simulink model "FMS"  (R2018b)
settings: configuration reference "fms_config" (kept outside this file)
values from neighbouring files (symbols this model uses):
  FMS_EXPORT = Simulink.Parameter(FMS_EXPORT_VALUE)    [fms_model_init.m]
  FMS_PARAM = Simulink.Parameter(FMS_PARAM_VALUE)    [fms_model_init.m]
undefined symbols (not defined in the file or in its folder): actuator_cmd, cmd_mask, ControlMode, ctrl_mode, DiscIntNeverNeededParam, FMS_Cmd, FMS_CONST, home, mode, PilotMode, r_cmd, reset, state, status, timestamp, u_cmd, VehicleState, VehicleStatus, wp_consume, wp_current
libraries: simulink x45, FMT_Model_Lib x35, hdlsllib x2
(part 2 of 3)

== system FMS/FMS Commander/Commander/Arm/Assist/Position/Position Command/Detect Movement ==
  FMS_In : Inport
  Abs1 : Abs
  Abs2 : Abs
  Bus Selector1 : BusSelector  OutputSignals=Pilot_Cmd.stick_roll,Pilot_Cmd.stick_throttle
  Compare To Constant : simulink/Logic and Bit Operations/Compare To Constant  relop=>  const=0.05  OutDataTypeStr=boolean
  Compare To Constant1 : simulink/Logic and Bit Operations/Compare To Constant  relop=<=  const=0.05  OutDataTypeStr=boolean
  Logical Operator : Logic  Operator=OR  AllPortsSameDT=off  OutDataTypeStr=boolean
  Motion State : Stateflow chart  TreatAsAtomicUnit=on
  motion_state : Outport
  wires:
  FMS_In/1 -> Bus Selector1/1
  Abs1/1 -> Compare To Constant/1
  Motion State/1(state) -> motion_state/1  "pos_ms"
  Bus Selector1/1 -> Abs1/1  "<stick_roll>"
  Compare To Constant1/1 -> Logical Operator/2
  Abs2/1 -> Compare To Constant1/1
  Bus Selector1/2 -> Abs2/1  "<stick_throttle>"
  Compare To Constant/1 -> Logical Operator/1
  Logical Operator/1 -> Motion State/1(motion_req)

== system FMS/FMS Commander/Commander/Arm/Assist/Position/Velocity_Command/DeadZone ==
  u : Inport
  Dead Zone : DeadZone  LowerValue=-th  UpperValue=th  SaturateOnIntegerOverflow=on
  Gain : Gain  Gain=1/(1-th)
  y : Outport
  wires:
  Gain/1 -> y/1
  Dead Zone/1 -> Gain/1
  u/1 -> Dead Zone/1

== system FMS/FMS Commander/Commander/Arm/Assist/Stabilize/Heading Command/Controller ==
  motion_state : Inport
  In Bus Element : Inport  Port=2  PortName=FMS_In
  In Bus Element1 : Inport  Port=2  PortName=FMS_In
  Brake Control : Subsystem  TreatAsAtomicUnit=on
  Hold Control : Subsystem  TreatAsAtomicUnit=on
  Merge : Merge  Inputs=3
  Move Control : Subsystem  TreatAsAtomicUnit=on
  Switch Case : SwitchCase  CaseConditions={MotionState.Hold, MotionState.Brake, MotionState.Move}  ShowDefaultCase=off
  psi_rate_cmd_radPs : Outport
  wires:
  Move Control/1(psi_rate_cmd_radPs) -> Merge/3
  Hold Control/1(psi_rate_cmd_radPs) -> Merge/1
  In Bus Element/1 -> Hold Control/1(FMS_In)
  Switch Case/1 -> Hold Control/Action
  motion_state/1 -> Switch Case/1
  In Bus Element1/1 -> Move Control/1(FMS_In)
  Merge/1 -> psi_rate_cmd_radPs/1
  Switch Case/3 -> Move Control/Action
  Brake Control/1(psi_rate_cmd_radPs) -> Merge/2
  Switch Case/2 -> Brake Control/Action

== system FMS/FMS Commander/Commander/Arm/Assist/Stabilize/Heading Command/Detect Movement ==
  FMS_In : Inport
  Abs1 : Abs
  Abs2 : Abs
  Bus Selector1 : BusSelector  OutputSignals=Pilot_Cmd.stick_roll,Pilot_Cmd.stick_throttle
  Compare To Constant : simulink/Logic and Bit Operations/Compare To Constant  relop=>  const=0.05  OutDataTypeStr=boolean
  Compare To Constant1 : simulink/Logic and Bit Operations/Compare To Constant  relop=<=  const=0.05  OutDataTypeStr=boolean
  Logical Operator : Logic  Operator=OR  AllPortsSameDT=off  OutDataTypeStr=boolean
  Motion State : Stateflow chart  TreatAsAtomicUnit=on
  motion_state : Outport
  wires:
  FMS_In/1 -> Bus Selector1/1
  Compare To Constant/1 -> Logical Operator/1
  Abs1/1 -> Compare To Constant/1
  Motion State/1(state) -> motion_state/1  "pos_ms"
  Bus Selector1/1 -> Abs1/1  "<stick_roll>"
  Bus Selector1/2 -> Abs2/1  "<stick_throttle>"
  Abs2/1 -> Compare To Constant1/1
  Compare To Constant1/1 -> Logical Operator/2
  Logical Operator/1 -> Motion State/1(motion_req)

== system FMS/FMS Commander/Commander/Arm/Auto/Mission/Mission_SubSystem/TD ==
  v : Inport
  Integrator : DiscreteIntegrator  SampleTime=-1  ICPrevOutput=DiscIntNeverNeededParam  ICPrevScaledInput=DiscIntNeverNeededParam
  Integrator1 : DiscreteIntegrator  SampleTime=-1  ICPrevOutput=DiscIntNeverNeededParam  ICPrevScaledInput=DiscIntNeverNeededParam
  Subtract : Sum  Inputs=+-
  "fhan " : Subsystem  mask{r0=2*9.806, h0=0.5}
      mask DialogControl ParameterGroupVar Prompt: fhan(v1,v2,r0,h0)
  v1 : Outport
  wires:
  "fhan "/1(fhan) -> Integrator/1
  Subtract/1 -> "fhan "/1(v1)
  Integrator/1 -> Integrator1/1, "fhan "/2(v2)  "v2"
  v/1 -> Subtract/2
  Integrator1/1 -> Subtract/1, v1/1

== system FMS/FMS Commander/Commander/Arm/Auto/Mission/Mission_SubSystem/Velocity Commander ==
  p1 : Inport
  p2 : Inport  Port=2
  p3 : Inport  Port=3
  L1 : Inport  Port=4
  In Bus Element : Inport  Port=5  PortName=FMS_In  Element=INS_Out.vn
  In Bus Element1 : Inport  Port=5  PortName=FMS_In  Element=INS_Out.ve
  AY_P : Gain  Gain=FMS_PARAM.AY_P
  L1 Reference WP : Subsystem
  Lateral Acceleration : Subsystem
  Mux1 : Mux  Inputs=2
  psi_rate_cmd : Outport
  wires:
  p3/1 -> Lateral Acceleration/3(p3), L1 Reference WP/3(P3)
  In Bus Element1/1 -> Mux1/2
  Mux1/1 -> Lateral Acceleration/1(Vg)
  p2/1 -> L1 Reference WP/2(P2)
  In Bus Element/1 -> Mux1/1
  L1 Reference WP/1(L1_WP) -> Lateral Acceleration/2(L1_WP)  "L1_WP"
  p1/1 -> L1 Reference WP/1(P1)
  L1/1 -> L1 Reference WP/4(L1), Lateral Acceleration/4(L1)
  Lateral Acceleration/1(l1_a_cmd) -> AY_P/1
  AY_P/1 -> psi_rate_cmd/1

== system FMS/FMS Commander/Commander/Arm/Auto/Mission/Mission_SubSystem/Way Points ==
  note: P1: path start point
      | P2: path end point
      | P3: vehicle point
  FMS_In : Inport
  Bus Selector : BusSelector  OutputSignals=INS_Out.x_R,INS_Out.y_R
  Bus Selector1 : BusSelector  OutputSignals=Cmd_In.sp_waypoint
  Bus Selector2 : BusSelector  OutputSignals=Cmd_In.cur_waypoint
  Mux : Mux  Inputs=2
  Reshape : Reshape  OutputDimensionality=Customize  OutputDimensions=[2,1]
  Reshape1 : Reshape  OutputDimensionality=Customize  OutputDimensions=[2,1]
  Reshape2 : Reshape  OutputDimensionality=Customize  OutputDimensions=[2,1]
  Selector : Selector  InputPortWidth=3  IndexOptions=Index vector (dialog)  Indices=[1 2]  OutputSizes=1
  Selector1 : Selector  InputPortWidth=3  IndexOptions=Index vector (dialog)  Indices=[1 2]  OutputSizes=1
  p1 : Outport
  p2 : Outport  Port=2
  p3 : Outport  Port=3
  wires:
  Reshape2/1 -> p3/1
  Reshape1/1 -> p1/1
  Reshape/1 -> p2/1
  Bus Selector/2 -> Mux/2  "<y_R>"
  Bus Selector/1 -> Mux/1  "<x_R>"
  Mux/1 -> Reshape2/1
  FMS_In/1 -> Bus Selector2/1, Bus Selector1/1, Bus Selector/1
  Bus Selector1/1 -> Selector/1  "<sp_waypoint>"
  Selector/1 -> Reshape/1
  Bus Selector2/1 -> Selector1/1  "<cur_waypoint>"
  Selector1/1 -> Reshape1/1

== system FMS/FMS Commander/Commander/Arm/Auto/Offboard/Rotation_Command/Heading_Control ==
  FMS_In : Inport
  Bus Selector1 : BusSelector  OutputSignals=Auto_Cmd.psi_cmd
  Bus Selector2 : BusSelector  OutputSignals=INS_Out.psi
  Gain2 : Gain  Gain=FMS_PARAM.YAW_P  OutDataTypeStr=single
  Sum : Sum  Inputs=-+|
  psi_err_saturation : Subsystem
  heading_r_cmd : Outport
  wires:
  Sum/1 -> psi_err_saturation/1(psi_err_in)  "psi_error_rad"
  psi_err_saturation/1(psi_err_rad) -> Gain2/1
  Gain2/1 -> heading_r_cmd/1
  FMS_In/1 -> Bus Selector1/1, Bus Selector2/1
  Bus Selector2/1 -> Sum/1  "<psi>"
  Bus Selector1/1 -> Sum/2  "<psi_cmd>"

== system FMS/FMS Commander/Commander/Arm/Auto/Offboard/Rotation_Command/Signal_Route ==
  FMS_In : Inport
  heading_r_cmd : Inport  Port=2
  pos_r_cmd : Inport  Port=3
  Bus Selector : BusSelector  OutputSignals=Auto_Cmd.cmd_mask
  Bus Selector1 : BusSelector  OutputSignals=Auto_Cmd.r_cmd
  Switch : Switch  Criteria=u2 > Threshold
  Switch1 : Switch  Criteria=u2 > Threshold
  psi_cmd_valid : simulink/Logic and Bit Operations/Bitwise Operator  logicop=AND  UseBitMask=on  BitMask=bin2dec('100000')  BitMaskRealWorld=Stored Integer
  r_cmd_valid : simulink/Logic and Bit Operations/Bitwise Operator  logicop=AND  UseBitMask=on  BitMask=bin2dec('100')  BitMaskRealWorld=Stored Integer
  r_cmd : Outport
  wires:
  FMS_In/1 -> Bus Selector1/1, Bus Selector/1
  pos_r_cmd/1 -> Switch1/3
  r_cmd_valid/1 -> Switch/2
  Bus Selector1/1 -> Switch/1  "<r_cmd>"
  Switch/1 -> r_cmd/1
  Bus Selector/1 -> psi_cmd_valid/1, r_cmd_valid/1  "<cmd_mask>"
  psi_cmd_valid/1 -> Switch1/2
  heading_r_cmd/1 -> Switch1/1
  Switch1/1 -> Switch/3

== system FMS/FMS Commander/Commander/Arm/Auto/Offboard/Rotation_Command/Velocity Commander ==
  p1 : Inport
  p2 : Inport  Port=2
  p3 : Inport  Port=3
  L1 : Inport  Port=4
  In Bus Element : Inport  Port=5  PortName=FMS_In  Element=INS_Out.vn
  In Bus Element1 : Inport  Port=5  PortName=FMS_In  Element=INS_Out.ve
  AccToRate : Gain  Gain=FMS_PARAM.AY_P
  L1 Reference WP : Subsystem
  Lateral Acceleration : Subsystem
  Mux1 : Mux  Inputs=2
  r_cmd : Outport
  wires:
  p3/1 -> Lateral Acceleration/3(p3), L1 Reference WP/3(P3)
  In Bus Element1/1 -> Mux1/2
  Mux1/1 -> Lateral Acceleration/1(Vg)
  p2/1 -> L1 Reference WP/2(P2)
  Lateral Acceleration/1(l1_a_cmd) -> AccToRate/1
  In Bus Element/1 -> Mux1/1
  L1 Reference WP/1(L1_WP) -> Lateral Acceleration/2(L1_WP)  "L1_WP"
  p1/1 -> L1 Reference WP/1(P1)
  L1/1 -> L1 Reference WP/4(L1), Lateral Acceleration/4(L1)
  AccToRate/1 -> r_cmd/1

== system FMS/FMS Commander/Commander/Arm/Auto/Offboard/Rotation_Command/Way Points ==
  note: P1: path start point
      | P2: path end point
      | P3: vehicle point
  FMS_In : Inport
  Bus Selector : BusSelector  OutputSignals=INS_Out.x_R,INS_Out.y_R
  Mux : Mux  Inputs=2
  Position_Control : Subsystem
  Reshape : Reshape  OutputDimensionality=Customize  OutputDimensions=[2,1]
  Reshape1 : Reshape  OutputDimensionality=Customize  OutputDimensions=[2,1]
  Reshape2 : Reshape  OutputDimensionality=Customize  OutputDimensions=[2,1]
  Selector : Selector  InputPortWidth=3  IndexOptions=Index vector (dialog)  Indices=[1 2]  OutputSizes=1
  p1 : Outport
  p2 : Outport  Port=2
  p3 : Outport  Port=3
  wires:
  Reshape2/1 -> p3/1
  Reshape1/1 -> p1/1
  Reshape/1 -> p2/1
  Bus Selector/2 -> Mux/2  "<y_R>"
  Bus Selector/1 -> Mux/1  "<x_R>"
  FMS_In/1 -> Position_Control/1(FMS_In), Bus Selector/1
  Selector/1 -> Reshape/1  "p2"
  Mux/1 -> Reshape2/1, Reshape1/1  "p1"
  Position_Control/1(pos_O_cmd) -> Selector/1

== system FMS/FMS Commander/Commander/Arm/Auto/Offboard/Velocity_Command/Command_Mask ==
  FMS_In : Inport
  Bus Selector1 : BusSelector  OutputSignals=Auto_Cmd.cmd_mask
  Compare To Zero2 : simulink/Logic and Bit Operations/Compare To Zero  relop=>  OutDataTypeStr=boolean
  u_cmd valid : simulink/Logic and Bit Operations/Bitwise Operator  logicop=AND  UseBitMask=on  BitMask=bin2dec('10000000000000')  BitMaskRealWorld=Stored Integer
  vel_mask : Outport
  wires:
  Compare To Zero2/1 -> vel_mask/1
  FMS_In/1 -> Bus Selector1/1
  u_cmd valid/1 -> Compare To Zero2/1
  Bus Selector1/1 -> u_cmd valid/1  "<cmd_mask>"

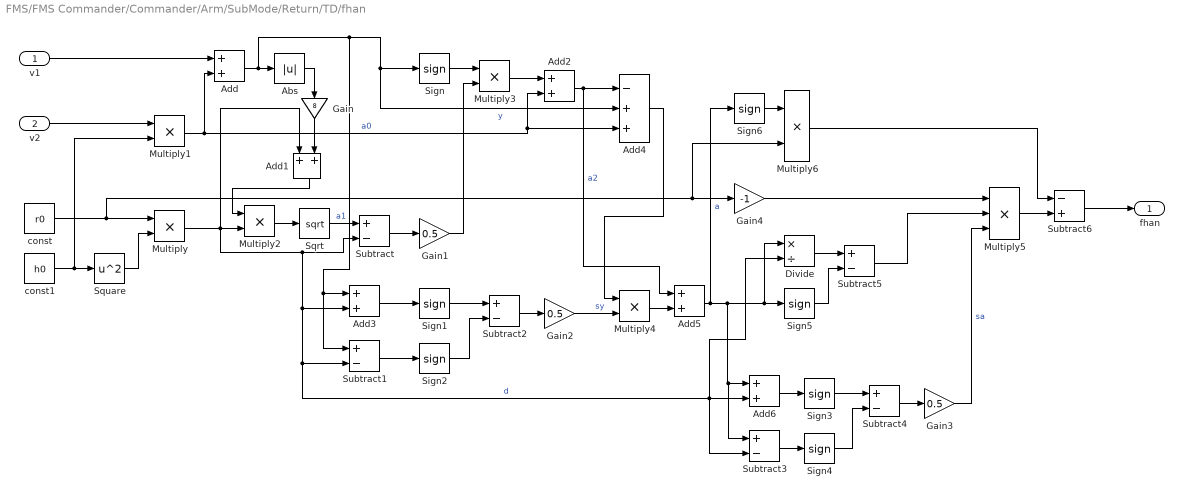
== system FMS/FMS Commander/Commander/Arm/SubMode/Return/TD/fhan  ==
  v1 : Inport
  v2 : Inport  Port=2
  Abs : Abs
  Add{,1..3,5..6} (6 alike) : Sum  OutDataTypeStr=Inherit: Same as first input
  Add4 : Sum  Inputs=-++
  Divide : Product  Inputs=*/
  Gain : Gain  Gain=8
  Gain1 : Gain  Gain=0.5  OutDataTypeStr=Inherit: Same as input
  Gain2 : Gain  Gain=0.5  OutDataTypeStr=Inherit: Same as input
  Gain3 : Gain  Gain=0.5  OutDataTypeStr=Inherit: Same as input
  Gain4 : Gain  Gain=-1  OutDataTypeStr=Inherit: Same as input
  Multiply{,1..3} (4 alike) : Product  OutDataTypeStr=Inherit: Same as first input
  Multiply4 : Product  OutDataTypeStr=single
  Multiply5 : Product  Inputs=3
  Multiply6 : Product  OutDataTypeStr=single
  Sign{,1..6} (7 alike) : Signum
  Sqrt : Sqrt  SaturateOnIntegerOverflow=on
  Square : Math  Operator=square  SaturateOnIntegerOverflow=on
  Subtract{,1..5} (6 alike) : Sum  Inputs=+-  OutDataTypeStr=Inherit: Same as first input
  Subtract6 : Sum  Inputs=-+  OutDataTypeStr=Inherit: Same as first input
  const : Constant  Value=r0  OutDataTypeStr=single
  const1 : Constant  Value=h0  OutDataTypeStr=single
  fhan : Outport
  wires:
  v1/1 -> Add/1
  Sign/1 -> Multiply3/1
  Gain2/1 -> Multiply4/2  "sy"
  v2/1 -> Multiply1/1
  Gain3/1 -> Multiply5/3  "sa"
  Subtract/1 -> Gain1/1
  Subtract6/1 -> fhan/1
  Sign2/1 -> Subtract2/2
  Sign4/1 -> Subtract4/2
  Abs/1 -> Gain/1
  Add4/1 -> Multiply4/1
  Sign5/1 -> Subtract5/2
  Sqrt/1 -> Subtract/1  "a1"
  Subtract3/1 -> Sign4/1
  Add1/1 -> Multiply2/1
  Subtract1/1 -> Sign2/1
  Divide/1 -> Subtract5/1
  Multiply3/1 -> Add2/1
  Gain/1 -> Add1/2
  const/1 -> Multiply6/2, Gain4/1, Multiply/1
  Add3/1 -> Sign1/1
  Subtract5/1 -> Multiply5/2
  Multiply4/1 -> Add5/2
  const1/1 -> Multiply1/2, Square/1
  Add5/1 -> Sign6/1, Sign5/1, Divide/1, Subtract3/1, Add6/1  "a"
  Multiply1/1 -> Add4/3, Add2/2, Add/2  "a0"
  Add/1 -> Subtract1/1, Add3/1, Add4/2, Sign/1, Abs/1  "y"
  Subtract2/1 -> Gain2/1
  Add2/1 -> Add4/1, Add5/1  "a2"
  Subtract4/1 -> Gain3/1
  Gain4/1 -> Multiply5/1
  Multiply5/1 -> Subtract6/2
  Sign6/1 -> Multiply6/1
  Sign3/1 -> Subtract4/1
  Add6/1 -> Sign3/1
  Multiply/1 -> Subtract/2, Divide/2, Subtract3/2, Add6/2, Subtract1/2, Add3/2, Add1/1, Multiply2/2  "d"
  Multiply6/1 -> Subtract6/1
  Gain1/1 -> Multiply3/2
  Square/1 -> Multiply/2
  Multiply2/1 -> Sqrt/1
  Sign1/1 -> Subtract2/1

== system FMS/FMS Commander/Commander/Arm/SubMode/Return/Velocity Commander/L1 Reference WP ==
  P1 : Inport
  P2 : Inport  Port=2
  P3 : Inport  Port=3
  L1 : Inport  Port=4
  Compare To Constant : simulink/Logic and Bit Operations/Compare To Constant  relop=>=  const=0  OutDataTypeStr=boolean
  Compare To Constant1 : simulink/Logic and Bit Operations/Compare To Constant  relop=>  const=0  OutDataTypeStr=boolean
  NearbyRefWP : MATLAB Function  TreatAsAtomicUnit=on
  OutRegionRegWP : MATLAB Function  TreatAsAtomicUnit=on
  Reshape : Reshape  OutputDimensionality=Customize  OutputDimensions=[2,1]
  SearchL1RefWP : MATLAB Function  TreatAsAtomicUnit=on
  Switch : Switch  Criteria=u2 > Threshold
  Switch1 : Switch  Criteria=u2 > Threshold
  L1_WP : Outport
  wires:
  Reshape/1 -> L1_WP/1
  Compare To Constant/1 -> Switch/2
  NearbyRefWP/2(d) -> Compare To Constant1/1  "distance"
  SearchL1RefWP/2(u) -> Compare To Constant/1  "l1_u"
  Compare To Constant1/1 -> Switch1/2
  P1/1 -> SearchL1RefWP/1(P1), OutRegionRegWP/1(P1)
  P2/1 -> SearchL1RefWP/2(P2), NearbyRefWP/1(P2), OutRegionRegWP/2(P2)
  P3/1 -> NearbyRefWP/2(P3), SearchL1RefWP/3(P3), OutRegionRegWP/3(P3)
  Switch/1 -> Switch1/3
  L1/1 -> SearchL1RefWP/4(L1), NearbyRefWP/3(L1)
  OutRegionRegWP/1(P) -> Switch/3  "out_WP"
  Switch1/1 -> Reshape/1
  SearchL1RefWP/1(P) -> Switch/1  "L1_Ref_P"
  NearbyRefWP/1(P) -> Switch1/1  "NearbyWP"

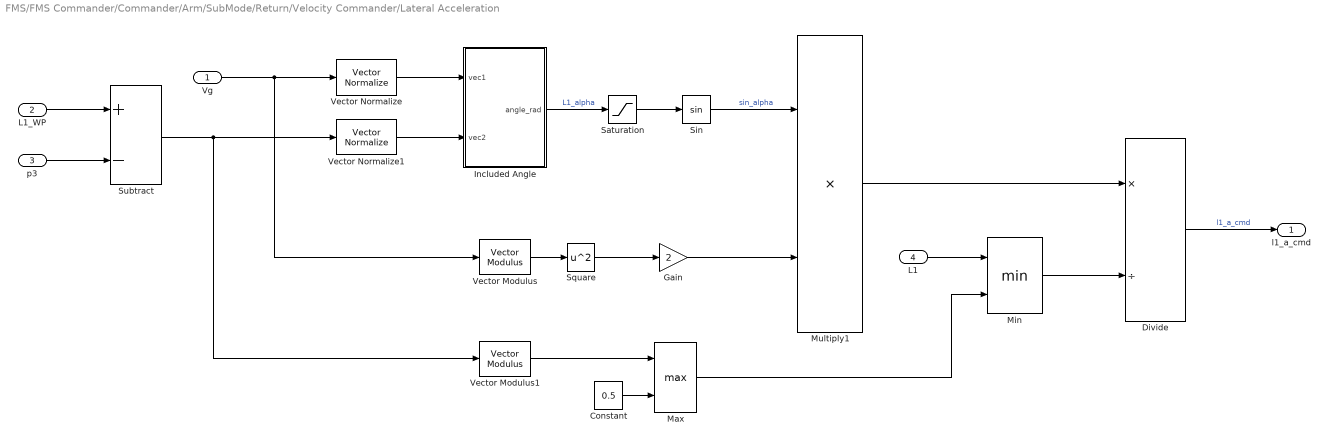
== system FMS/FMS Commander/Commander/Arm/SubMode/Return/Velocity Commander/Lateral Acceleration ==
  Vg : Inport
  L1_WP : Inport  Port=2
  p3 : Inport  Port=3
  L1 : Inport  Port=4
  Constant : Constant  Value=0.5  OutDataTypeStr=Inherit: Inherit via back propagation
  Divide : Product  Inputs=*/
  Gain : Gain  Gain=2
  Included Angle : Subsystem
  Max : MinMax  Function=max  Inputs=2
  Min : MinMax  Inputs=2
  Multiply1 : Product
  Saturation : Saturate  UpperLimit=pi/2  LowerLimit=-pi/2
  Sin : Trigonometry
  Square : Math  Operator=square  SaturateOnIntegerOverflow=on
  Subtract : Sum  Inputs=+-
  Vector Modulus : FMT_Model_Lib/Math/Vector Modulus
      settings: SourceProductName=FMT Toolbox
  Vector Modulus1 : FMT_Model_Lib/Math/Vector Modulus
      settings: SourceProductName=FMT Toolbox
  Vector Normalize : FMT_Model_Lib/Math/Vector Normalize
      settings: SourceProductName=FMT Toolbox
  Vector Normalize1 : FMT_Model_Lib/Math/Vector Normalize
      settings: SourceProductName=FMT Toolbox
  l1_a_cmd : Outport
  wires:
  Saturation/1 -> Sin/1
  Included Angle/1(angle_rad) -> Saturation/1  "L1_alpha"
  Vector Modulus/1 -> Square/1
  Subtract/1 -> Vector Modulus1/1, Vector Normalize1/1
  Gain/1 -> Multiply1/2
  L1_WP/1 -> Subtract/1
  Vector Normalize/1 -> Included Angle/1(vec1)
  Multiply1/1 -> Divide/1
  Divide/1 -> l1_a_cmd/1  "l1_a_cmd"
  Vector Normalize1/1 -> Included Angle/2(vec2)
  Square/1 -> Gain/1
  L1/1 -> Min/1
  Vg/1 -> Vector Normalize/1, Vector Modulus/1
  Sin/1 -> Multiply1/1  "sin_alpha"
  p3/1 -> Subtract/2
  Vector Modulus1/1 -> Max/1
  Constant/1 -> Max/2
  Max/1 -> Min/2
  Min/1 -> Divide/2

== system FMS/FMS Commander/Commander/Arm/Assist/Position/Position Command/Controller/Brake Control ==
  Action Port : ActionPort  InitializeStates=reset  ActionType=case
  Constant : Constant  Value=0  OutDataTypeStr=single
  psi_rate_cmd_radPs : Outport
  wires:
  Constant/1 -> psi_rate_cmd_radPs/1

== system FMS/FMS Commander/Commander/Arm/Assist/Position/Position Command/Controller/Hold Control ==
  FMS_In : Inport
  u_cmd : Inport  Port=2
  Action Port : ActionPort  InitializeStates=reset  ActionType=case
  AY_P : Gain  Gain=FMS_PARAM.AY_P
  Bus Selector1 : BusSelector  OutputSignals=INS_Out.vn,INS_Out.ve
  FMS_In1 : InportShadow
  L1 : Constant  Value=FMS_PARAM.L1  OutDataTypeStr=single
  L1_Reference_WP : Subsystem
  Lateral_Acceleration : Subsystem
  Mux : Mux  Inputs=2
  Path_Ray : Subsystem
  psi_rate_cmd_radPs : Outport
  wires:
  FMS_In/1 -> Path_Ray/1(FMS_In)
  Path_Ray/1(p_vehicle) -> Lateral_Acceleration/1(p_vehicle), L1_Reference_WP/1(c)
  Path_Ray/2(p_0) -> L1_Reference_WP/2(p_0)
  Path_Ray/3(n) -> L1_Reference_WP/3(n)
  L1/1 -> L1_Reference_WP/4(L1), Lateral_Acceleration/3(L1)
  FMS_In1/1 -> Bus Selector1/1
  Bus Selector1/1 -> Mux/1  "<vn>"
  Bus Selector1/2 -> Mux/2  "<ve>"
  L1_Reference_WP/1(L1_WP) -> Lateral_Acceleration/2(L1_WP)
  Mux/1 -> Lateral_Acceleration/4(Vg)
  Lateral_Acceleration/1(ay_cmd_mPs2) -> AY_P/1
  u_cmd/1 -> Path_Ray/2(u_cmd)
  AY_P/1 -> psi_rate_cmd_radPs/1

== system FMS/FMS Commander/Commander/Arm/Assist/Position/Position Command/Controller/Move Control ==
  FMS_In : Inport
  Action Port : ActionPort  InitializeStates=reset  ActionType=case
  Bus Selector : BusSelector  OutputSignals=Pilot_Cmd.stick_roll
  DeadZone : Subsystem  mask{th=0.05}
      mask prompts: th "Threshold"
      mask Display: disp('Dead Zone')
  Gain : Gain  Gain=FMS_PARAM.MAX_PSI_RATE
  psi_rate_cmd_radPs : Outport
  wires:
  Bus Selector/1 -> DeadZone/1(u)  "<stick_roll>"
  FMS_In/1 -> Bus Selector/1
  DeadZone/1(y) -> Gain/1
  Gain/1 -> psi_rate_cmd_radPs/1

== system FMS/FMS Commander/Commander/Arm/Assist/Stabilize/Heading Command/Controller/Brake Control ==
  Action Port : ActionPort  InitializeStates=reset  ActionType=case
  Constant : Constant  Value=0  OutDataTypeStr=single
  psi_rate_cmd_radPs : Outport
  wires:
  Constant/1 -> psi_rate_cmd_radPs/1

== system FMS/FMS Commander/Commander/Arm/Assist/Stabilize/Heading Command/Controller/Hold Control ==
  FMS_In : Inport
  Action Port : ActionPort  InitializeStates=reset  ActionType=case
  Bus_Selection : Subsystem
  Delay : Delay  DelayLength=1  InitialConditionSource=Input port
      settings: InputPortMap=u0,p4
  Gain2 : Gain  Gain=FMS_PARAM.YAW_P  OutDataTypeStr=single
  Sum : Sum  Inputs=-+|
  psi_err_saturation : Subsystem
  psi_rate_cmd_radPs : Outport
  wires:
  FMS_In/1 -> Bus_Selection/1(FMS_In)
  Gain2/1 -> psi_rate_cmd_radPs/1
  psi_err_saturation/1(psi_err_rad) -> Gain2/1
  Sum/1 -> psi_err_saturation/1(psi_err_in)  "psi_error_rad"
  Delay/1 -> Sum/2, Delay/1  "psi_cmd_rad"
  Bus_Selection/1(psi_rad) -> Delay/2, Sum/1  "psi_est_rad"

== system FMS/FMS Commander/Commander/Arm/Assist/Stabilize/Heading Command/Controller/Move Control ==
  FMS_In : Inport
  Action Port : ActionPort  InitializeStates=reset  ActionType=case
  Bus Selector : BusSelector  OutputSignals=Pilot_Cmd.stick_roll
  DeadZone : Subsystem  mask{th=0.05}
      mask prompts: th "Threshold"
      mask Display: disp('Dead Zone')
  Gain : Gain  Gain=FMS_PARAM.MAX_PSI_RATE
  psi_rate_cmd_radPs : Outport
  wires:
  Bus Selector/1 -> DeadZone/1(u)  "<stick_roll>"
  FMS_In/1 -> Bus Selector/1
  DeadZone/1(y) -> Gain/1
  Gain/1 -> psi_rate_cmd_radPs/1

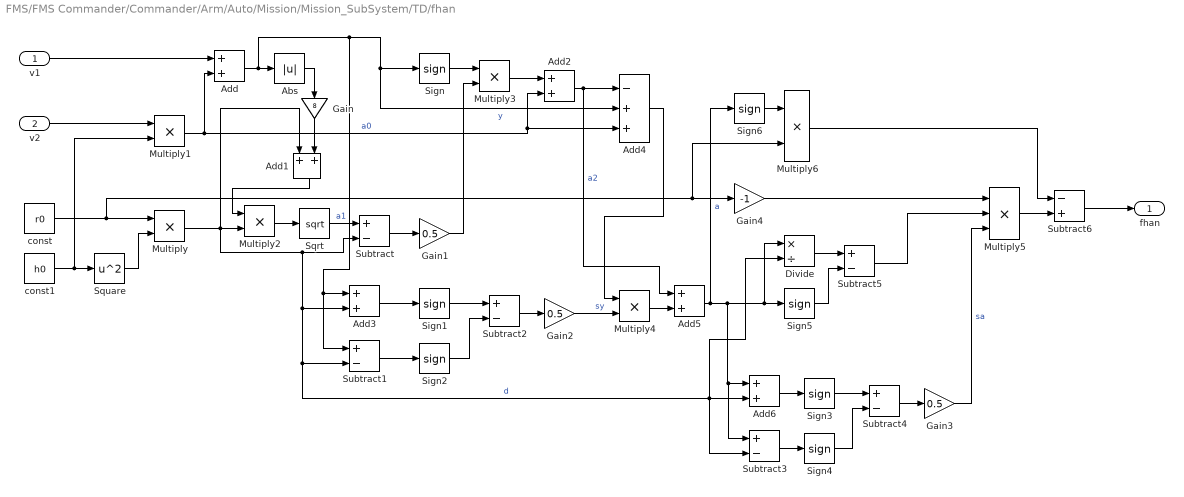
== system FMS/FMS Commander/Commander/Arm/Auto/Mission/Mission_SubSystem/TD/fhan  ==
  v1 : Inport
  v2 : Inport  Port=2
  Abs : Abs
  Add{,1..3,5..6} (6 alike) : Sum  OutDataTypeStr=Inherit: Same as first input
  Add4 : Sum  Inputs=-++
  Divide : Product  Inputs=*/
  Gain : Gain  Gain=8
  Gain1 : Gain  Gain=0.5  OutDataTypeStr=Inherit: Same as input
  Gain2 : Gain  Gain=0.5  OutDataTypeStr=Inherit: Same as input
  Gain3 : Gain  Gain=0.5  OutDataTypeStr=Inherit: Same as input
  Gain4 : Gain  Gain=-1  OutDataTypeStr=Inherit: Same as input
  Multiply{,1..3} (4 alike) : Product  OutDataTypeStr=Inherit: Same as first input
  Multiply4 : Product  OutDataTypeStr=single
  Multiply5 : Product  Inputs=3
  Multiply6 : Product  OutDataTypeStr=single
  Sign{,1..6} (7 alike) : Signum
  Sqrt : Sqrt  SaturateOnIntegerOverflow=on
  Square : Math  Operator=square  SaturateOnIntegerOverflow=on
  Subtract{,1..5} (6 alike) : Sum  Inputs=+-  OutDataTypeStr=Inherit: Same as first input
  Subtract6 : Sum  Inputs=-+  OutDataTypeStr=Inherit: Same as first input
  const : Constant  Value=r0  OutDataTypeStr=single
  const1 : Constant  Value=h0  OutDataTypeStr=single
  fhan : Outport
  wires:
  v1/1 -> Add/1
  Sign/1 -> Multiply3/1
  Gain2/1 -> Multiply4/2  "sy"
  v2/1 -> Multiply1/1
  Gain3/1 -> Multiply5/3  "sa"
  Subtract/1 -> Gain1/1
  Subtract6/1 -> fhan/1
  Sign2/1 -> Subtract2/2
  Sign4/1 -> Subtract4/2
  Abs/1 -> Gain/1
  Add4/1 -> Multiply4/1
  Sign5/1 -> Subtract5/2
  Sqrt/1 -> Subtract/1  "a1"
  Subtract3/1 -> Sign4/1
  Add1/1 -> Multiply2/1
  Subtract1/1 -> Sign2/1
  Divide/1 -> Subtract5/1
  Multiply3/1 -> Add2/1
  Gain/1 -> Add1/2
  const/1 -> Multiply6/2, Gain4/1, Multiply/1
  Add3/1 -> Sign1/1
  Subtract5/1 -> Multiply5/2
  Multiply4/1 -> Add5/2
  const1/1 -> Multiply1/2, Square/1
  Add5/1 -> Sign6/1, Sign5/1, Divide/1, Subtract3/1, Add6/1  "a"
  Multiply1/1 -> Add4/3, Add2/2, Add/2  "a0"
  Add/1 -> Subtract1/1, Add3/1, Add4/2, Sign/1, Abs/1  "y"
  Subtract2/1 -> Gain2/1
  Add2/1 -> Add4/1, Add5/1  "a2"
  Subtract4/1 -> Gain3/1
  Gain4/1 -> Multiply5/1
  Multiply5/1 -> Subtract6/2
  Sign6/1 -> Multiply6/1
  Sign3/1 -> Subtract4/1
  Add6/1 -> Sign3/1
  Multiply/1 -> Subtract/2, Divide/2, Subtract3/2, Add6/2, Subtract1/2, Add3/2, Add1/1, Multiply2/2  "d"
  Multiply6/1 -> Subtract6/1
  Gain1/1 -> Multiply3/2
  Square/1 -> Multiply/2
  Multiply2/1 -> Sqrt/1
  Sign1/1 -> Subtract2/1

== system FMS/FMS Commander/Commander/Arm/Auto/Mission/Mission_SubSystem/Velocity Commander/L1 Reference WP ==
  P1 : Inport
  P2 : Inport  Port=2
  P3 : Inport  Port=3
  L1 : Inport  Port=4
  Compare To Constant : simulink/Logic and Bit Operations/Compare To Constant  relop=>=  const=0  OutDataTypeStr=boolean
  Compare To Constant1 : simulink/Logic and Bit Operations/Compare To Constant  relop=>  const=0  OutDataTypeStr=boolean
  NearbyRefWP : MATLAB Function  TreatAsAtomicUnit=on
  OutRegionRegWP : MATLAB Function  TreatAsAtomicUnit=on
  Reshape : Reshape  OutputDimensionality=Customize  OutputDimensions=[2,1]
  SearchL1RefWP : MATLAB Function  TreatAsAtomicUnit=on
  Switch : Switch  Criteria=u2 > Threshold
  Switch1 : Switch  Criteria=u2 > Threshold
  L1_WP : Outport
  wires:
  Reshape/1 -> L1_WP/1
  Compare To Constant/1 -> Switch/2
  NearbyRefWP/2(d) -> Compare To Constant1/1  "distance"
  SearchL1RefWP/2(u) -> Compare To Constant/1  "l1_u"
  Compare To Constant1/1 -> Switch1/2
  P1/1 -> SearchL1RefWP/1(P1), OutRegionRegWP/1(P1)
  P2/1 -> SearchL1RefWP/2(P2), NearbyRefWP/1(P2), OutRegionRegWP/2(P2)
  P3/1 -> NearbyRefWP/2(P3), SearchL1RefWP/3(P3), OutRegionRegWP/3(P3)
  Switch/1 -> Switch1/3
  L1/1 -> SearchL1RefWP/4(L1), NearbyRefWP/3(L1)
  OutRegionRegWP/1(P) -> Switch/3  "out_WP"
  Switch1/1 -> Reshape/1
  SearchL1RefWP/1(P) -> Switch/1  "L1_Ref_P"
  NearbyRefWP/1(P) -> Switch1/1  "NearbyWP"

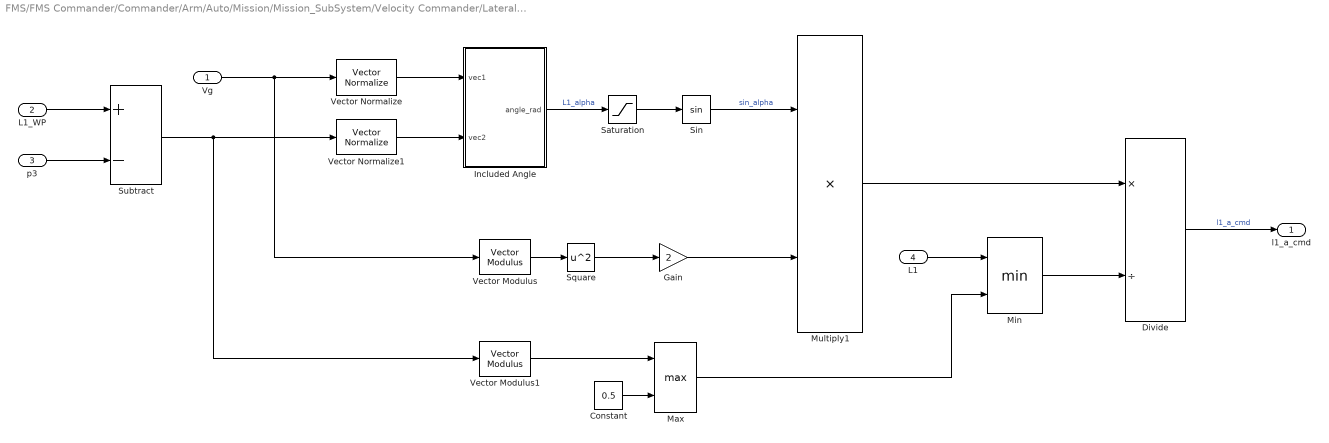
== system FMS/FMS Commander/Commander/Arm/Auto/Mission/Mission_SubSystem/Velocity Commander/Lateral Acceleration ==
  Vg : Inport
  L1_WP : Inport  Port=2
  p3 : Inport  Port=3
  L1 : Inport  Port=4
  Constant : Constant  Value=0.5  OutDataTypeStr=Inherit: Inherit via back propagation
  Divide : Product  Inputs=*/
  Gain : Gain  Gain=2
  Included Angle : Subsystem
  Max : MinMax  Function=max  Inputs=2
  Min : MinMax  Inputs=2
  Multiply1 : Product
  Saturation : Saturate  UpperLimit=pi/2  LowerLimit=-pi/2
  Sin : Trigonometry
  Square : Math  Operator=square  SaturateOnIntegerOverflow=on
  Subtract : Sum  Inputs=+-
  Vector Modulus : FMT_Model_Lib/Math/Vector Modulus
      settings: SourceProductName=FMT Toolbox
  Vector Modulus1 : FMT_Model_Lib/Math/Vector Modulus
      settings: SourceProductName=FMT Toolbox
  Vector Normalize : FMT_Model_Lib/Math/Vector Normalize
      settings: SourceProductName=FMT Toolbox
  Vector Normalize1 : FMT_Model_Lib/Math/Vector Normalize
      settings: SourceProductName=FMT Toolbox
  l1_a_cmd : Outport
  wires:
  Saturation/1 -> Sin/1
  Included Angle/1(angle_rad) -> Saturation/1  "L1_alpha"
  Vector Modulus/1 -> Square/1
  Subtract/1 -> Vector Modulus1/1, Vector Normalize1/1
  Gain/1 -> Multiply1/2
  L1_WP/1 -> Subtract/1
  Vector Normalize/1 -> Included Angle/1(vec1)
  Multiply1/1 -> Divide/1
  Divide/1 -> l1_a_cmd/1  "l1_a_cmd"
  Vector Normalize1/1 -> Included Angle/2(vec2)
  Square/1 -> Gain/1
  L1/1 -> Min/1
  Vg/1 -> Vector Normalize/1, Vector Modulus/1
  Sin/1 -> Multiply1/1  "sin_alpha"
  p3/1 -> Subtract/2
  Vector Modulus1/1 -> Max/1
  Constant/1 -> Max/2
  Max/1 -> Min/2
  Min/1 -> Divide/2

== system FMS/FMS Commander/Commander/Arm/Auto/Offboard/Rotation_Command/Heading_Control/psi_err_saturation ==
  psi_err_in : Inport
  Abs : Abs
  Compare To Constant : simulink/Logic and Bit Operations/Compare To Constant  relop=>  const=pi  OutDataTypeStr=boolean
  Constant : Constant  Value=2*pi  OutDataTypeStr=single
  Multiply : Product
  Sign : Signum
  Subtract : Sum  Inputs=-+
  Switch : Switch  Criteria=u2 > Threshold
  psi_err_rad : Outport
  wires:
  Multiply/1 -> Switch/1
  Sign/1 -> Multiply/2
  Subtract/1 -> Multiply/1
  Constant/1 -> Subtract/1
  Switch/1 -> psi_err_rad/1
  Compare To Constant/1 -> Switch/2
  Abs/1 -> Compare To Constant/1, Subtract/2
  psi_err_in/1 -> Abs/1, Switch/3, Sign/1

== system FMS/FMS Commander/Commander/Arm/Auto/Offboard/Rotation_Command/Velocity Commander/L1 Reference WP ==
  P1 : Inport
  P2 : Inport  Port=2
  P3 : Inport  Port=3
  L1 : Inport  Port=4
  Compare To Constant : simulink/Logic and Bit Operations/Compare To Constant  relop=>=  const=0  OutDataTypeStr=boolean
  Compare To Constant1 : simulink/Logic and Bit Operations/Compare To Constant  relop=>  const=0  OutDataTypeStr=boolean
  NearbyRefWP : MATLAB Function  TreatAsAtomicUnit=on
  OutRegionRegWP : MATLAB Function  TreatAsAtomicUnit=on
  Reshape : Reshape  OutputDimensionality=Customize  OutputDimensions=[2,1]
  SearchL1RefWP : MATLAB Function  TreatAsAtomicUnit=on
  Switch : Switch  Criteria=u2 > Threshold
  Switch1 : Switch  Criteria=u2 > Threshold
  L1_WP : Outport
  wires:
  Reshape/1 -> L1_WP/1
  Compare To Constant/1 -> Switch/2
  NearbyRefWP/2(d) -> Compare To Constant1/1  "distance"
  SearchL1RefWP/2(u) -> Compare To Constant/1  "l1_u"
  Compare To Constant1/1 -> Switch1/2
  P1/1 -> SearchL1RefWP/1(P1), OutRegionRegWP/1(P1)
  P2/1 -> SearchL1RefWP/2(P2), NearbyRefWP/1(P2), OutRegionRegWP/2(P2)
  P3/1 -> NearbyRefWP/2(P3), SearchL1RefWP/3(P3), OutRegionRegWP/3(P3)
  Switch/1 -> Switch1/3
  L1/1 -> SearchL1RefWP/4(L1), NearbyRefWP/3(L1)
  OutRegionRegWP/1(P) -> Switch/3  "out_WP"
  Switch1/1 -> Reshape/1
  SearchL1RefWP/1(P) -> Switch/1  "L1_Ref_P"
  NearbyRefWP/1(P) -> Switch1/1  "NearbyWP"

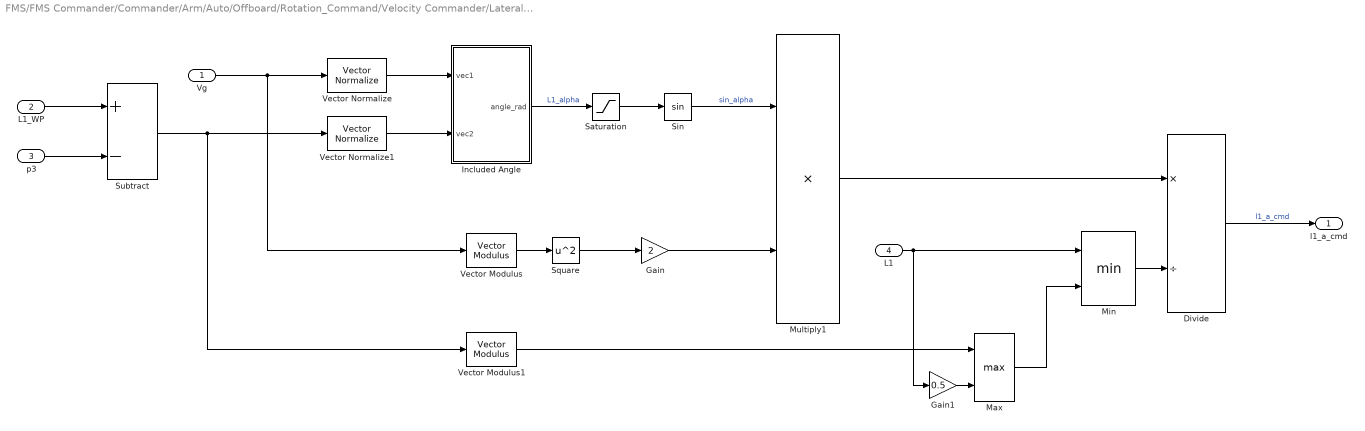
== system FMS/FMS Commander/Commander/Arm/Auto/Offboard/Rotation_Command/Velocity Commander/Lateral Acceleration ==
  Vg : Inport
  L1_WP : Inport  Port=2
  p3 : Inport  Port=3
  L1 : Inport  Port=4
  Divide : Product  Inputs=*/
  Gain : Gain  Gain=2
  Gain1 : Gain  Gain=0.5
  Included Angle : Subsystem
  Max : MinMax  Function=max  Inputs=2
  Min : MinMax  Inputs=2
  Multiply1 : Product
  Saturation : Saturate  UpperLimit=pi/2  LowerLimit=-pi/2
  Sin : Trigonometry
  Square : Math  Operator=square  SaturateOnIntegerOverflow=on
  Subtract : Sum  Inputs=+-
  Vector Modulus : FMT_Model_Lib/Math/Vector Modulus
      settings: SourceProductName=FMT Toolbox
  Vector Modulus1 : FMT_Model_Lib/Math/Vector Modulus
      settings: SourceProductName=FMT Toolbox
  Vector Normalize : FMT_Model_Lib/Math/Vector Normalize
      settings: SourceProductName=FMT Toolbox
  Vector Normalize1 : FMT_Model_Lib/Math/Vector Normalize
      settings: SourceProductName=FMT Toolbox
  l1_a_cmd : Outport
  wires:
  Saturation/1 -> Sin/1
  Included Angle/1(angle_rad) -> Saturation/1  "L1_alpha"
  Vector Modulus/1 -> Square/1
  Subtract/1 -> Vector Modulus1/1, Vector Normalize1/1
  Gain/1 -> Multiply1/2
  L1_WP/1 -> Subtract/1
  Vector Normalize/1 -> Included Angle/1(vec1)
  Multiply1/1 -> Divide/1
  Divide/1 -> l1_a_cmd/1  "l1_a_cmd"
  Vector Normalize1/1 -> Included Angle/2(vec2)
  Square/1 -> Gain/1
  L1/1 -> Gain1/1, Min/1
  Vg/1 -> Vector Normalize/1, Vector Modulus/1
  Sin/1 -> Multiply1/1  "sin_alpha"
  p3/1 -> Subtract/2
  Vector Modulus1/1 -> Max/1
  Max/1 -> Min/2
  Min/1 -> Divide/2
  Gain1/1 -> Max/2

== system FMS/FMS Commander/Commander/Arm/Auto/Offboard/Rotation_Command/Way Points/Position_Control ==
  FMS_In : Inport
  Body_FRD : Subsystem
  Bus Selector : BusSelector  OutputSignals=INS_Out.psi
  Bus Selector2 : BusSelector  OutputSignals=Auto_Cmd.frame
  Command_Mask : Subsystem
  Global_NED : Subsystem
  Index Vector : MultiPortSwitch  DataPortOrder=Zero-based contiguous  Inputs=4  zeroidx=on
  Local_FRD : Subsystem
  Local_NED : Subsystem
  Position_Command : Subsystem
  pos_O_cmd : Outport
  wires:
  Position_Command/1(pos_cmd_R) -> Local_FRD/1(pos_R_cmd), Body_FRD/2(pos_B_cmd), Local_NED/1(pos_R_cmd), Global_NED/1(pos_O_cmd)
  Bus Selector/1 -> Body_FRD/1(psi)  "<psi>"
  Bus Selector2/1 -> Index Vector/1  "<frame>"
  FMS_In/1 -> Position_Command/1(FMS_In), Bus Selector2/1, Bus Selector/1, Command_Mask/1(FMS_In)
  Command_Mask/1(pos_mask) -> Body_FRD/3(pos_mask), Local_FRD/2(pos_mask), Local_NED/2(pos_mask), Global_NED/2(pos_mask)
  Global_NED/1(pos_cmd) -> Index Vector/2
  Index Vector/1 -> pos_O_cmd/1
  Body_FRD/1(pos_O_cmd) -> Index Vector/5
  Local_FRD/1(pos_O_cmd) -> Index Vector/4
  Local_NED/1(pos_O_cmd) -> Index Vector/3

== system FMS/FMS Commander/Commander/Arm/SubMode/Return/Velocity Commander/Lateral Acceleration/Included Angle ==
  vec1 : Inport
  vec2 : Inport  Port=2
  2D Cross Product : FMT_Model_Lib/Math/2D Cross Product
      settings: SourceProductName=FMT Toolbox
  Acos : Trigonometry  Operator=acos
  Constant4 : Constant  OutDataTypeStr=single
  Demux : Demux  Outputs=2
  Demux1 : Demux  Outputs=2
  Dot Product : DotProduct  InputSameDT=on  OutDataTypeStr=Inherit: Inherit via internal rule
  Multiply : Product
  Mux : Mux  Inputs=2
  Mux1 : Mux  Inputs=2
  Sign1 : Signum
  Switch2 : Switch  Criteria=u2 ~= 0
  Vector Normalize : FMT_Model_Lib/Math/Vector Normalize
      settings: SourceProductName=FMT Toolbox
  Vector Normalize1 : FMT_Model_Lib/Math/Vector Normalize
      settings: SourceProductName=FMT Toolbox
  angle_rad : Outport
  wires:
  Switch2/1 -> Multiply/2
  Acos/1 -> Multiply/1
  Mux/1 -> Vector Normalize1/1
  vec2/1 -> Demux/1
  Constant4/1 -> Switch2/3
  Demux/1 -> Mux/2
  vec1/1 -> Demux1/1
  Multiply/1 -> angle_rad/1
  2D Cross Product/1 -> Sign1/1
  Vector Normalize/1 -> 2D Cross Product/2, Dot Product/1
  Demux/2 -> Mux/1
  Vector Normalize1/1 -> 2D Cross Product/1, Dot Product/2
  Sign1/1 -> Switch2/2, Switch2/1
  Demux1/2 -> Mux1/1
  Mux1/1 -> Vector Normalize/1
  Demux1/1 -> Mux1/2
  Dot Product/1 -> Acos/1

== system FMS/FMS Commander/Commander/Arm/Assist/Position/Position Command/Controller/Hold Control/L1_Reference_WP ==
  c : Inport
  p_0 : Inport  Port=2
  n : Inport  Port=3
  L1 : Inport  Port=4
  Compare To Zero : simulink/Logic and Bit Operations/Compare To Zero  relop=>  OutDataTypeStr=boolean
  OutRegionRefWP : MATLAB Function  TreatAsAtomicUnit=on
  SearchL1RefWP : MATLAB Function  TreatAsAtomicUnit=on
  Switch : Switch  Criteria=u2 > Threshold
  L1_WP : Outport
  wires:
  c/1 -> OutRegionRefWP/1(c), SearchL1RefWP/1(c)
  p_0/1 -> OutRegionRefWP/2(p0), SearchL1RefWP/2(p0)
  n/1 -> OutRegionRefWP/3(n), SearchL1RefWP/3(n)  "L1_n"
  L1/1 -> SearchL1RefWP/4(L1)
  SearchL1RefWP/1(P) -> Switch/1
  SearchL1RefWP/2(t) -> Compare To Zero/1  "L1_t"
  Compare To Zero/1 -> Switch/2
  OutRegionRefWP/1(P) -> Switch/3
  Switch/1 -> L1_WP/1  "L1_WP"

== system FMS/FMS Commander/Commander/Arm/Assist/Position/Position Command/Controller/Hold Control/Lateral_Acceleration ==
  p_vehicle : Inport
  L1_WP : Inport  Port=2
  L1 : Inport  Port=3
  Vg : Inport  Port=4
  L1_Lateral_Acceleration : Subsystem
  Subtract : Sum  Inputs=+-
  ay_cmd_mPs2 : Outport
  wires:
  L1_WP/1 -> Subtract/1  "l1_wp2"
  p_vehicle/1 -> Subtract/2
  L1/1 -> L1_Lateral_Acceleration/1(L1)
  Vg/1 -> L1_Lateral_Acceleration/2(Vg)
  Subtract/1 -> L1_Lateral_Acceleration/3(l1_path)  "l1_path"
  L1_Lateral_Acceleration/1(l1_a_cmd) -> ay_cmd_mPs2/1

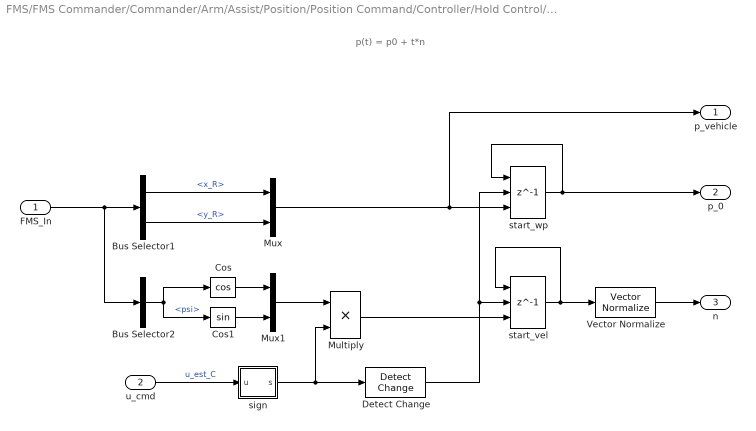
== system FMS/FMS Commander/Commander/Arm/Assist/Position/Position Command/Controller/Hold Control/Path_Ray ==
  note: p(t) = p0 + t*n
  FMS_In : Inport
  u_cmd : Inport  Port=2
  Bus Selector1 : BusSelector  OutputSignals=INS_Out.x_R,INS_Out.y_R
  Bus Selector2 : BusSelector  OutputSignals=INS_Out.psi
  Cos : Trigonometry  Operator=cos
  Cos1 : Trigonometry
  Detect Change : simulink/Logic and Bit Operations/Detect Change  vinit=0  OutDataTypeStr=boolean
  Multiply : Product
  Mux : Mux  Inputs=2
  Mux1 : Mux  Inputs=2
  Vector Normalize : FMT_Model_Lib/Math/Vector Normalize
      settings: SourceProductName=FMT Toolbox
  sign : Subsystem
  start_vel : Delay  DelayLength=1  InitialConditionSource=Input port  ExternalReset=Rising
      settings: InputPortMap=u0,r5,p4
  start_wp : Delay  DelayLength=1  InitialConditionSource=Input port  ExternalReset=Rising
      settings: InputPortMap=u0,r5,p4
  p_vehicle : Outport
  p_0 : Outport  Port=2
  n : Outport  Port=3
  wires:
  Bus Selector1/2 -> Mux/2  "<y_R>"
  Mux/1 -> p_vehicle/1, start_wp/3
  start_wp/1 -> start_wp/1, p_0/1
  Bus Selector1/1 -> Mux/1  "<x_R>"
  start_vel/1 -> start_vel/1, Vector Normalize/1
  Vector Normalize/1 -> n/1
  FMS_In/1 -> Bus Selector2/1, Bus Selector1/1
  Detect Change/1 -> start_wp/2, start_vel/2
  Cos/1 -> Mux1/1
  Bus Selector2/1 -> Cos1/1, Cos/1  "<psi>"
  Cos1/1 -> Mux1/2
  u_cmd/1 -> sign/1(u)  "u_est_C"
  sign/1(s) -> Multiply/2, Detect Change/1
  Mux1/1 -> Multiply/1
  Multiply/1 -> start_vel/3

== system FMS/FMS Commander/Commander/Arm/Assist/Position/Position Command/Controller/Move Control/DeadZone ==
  u : Inport
  Dead Zone : DeadZone  LowerValue=-th  UpperValue=th  SaturateOnIntegerOverflow=on
  Gain : Gain  Gain=1/(1-th)
  y : Outport
  wires:
  Gain/1 -> y/1
  Dead Zone/1 -> Gain/1
  u/1 -> Dead Zone/1

== system FMS/FMS Commander/Commander/Arm/Assist/Stabilize/Heading Command/Controller/Hold Control/Bus_Selection ==
  FMS_In : Inport
  Bus Selector2 : BusSelector  OutputSignals=INS_Out.psi
  psi_rad : Outport
  wires:
  Bus Selector2/1 -> psi_rad/1  "<psi>"
  FMS_In/1 -> Bus Selector2/1

== system FMS/FMS Commander/Commander/Arm/Assist/Stabilize/Heading Command/Controller/Hold Control/psi_err_saturation ==
  psi_err_in : Inport
  Abs : Abs
  Compare To Constant : simulink/Logic and Bit Operations/Compare To Constant  relop=>  const=pi  OutDataTypeStr=boolean
  Constant : Constant  Value=2*pi  OutDataTypeStr=single
  Multiply : Product
  Sign : Signum
  Subtract : Sum  Inputs=-+
  Switch : Switch  Criteria=u2 > Threshold
  psi_err_rad : Outport
  wires:
  Multiply/1 -> Switch/1
  Sign/1 -> Multiply/2
  Subtract/1 -> Multiply/1
  Constant/1 -> Subtract/1
  Switch/1 -> psi_err_rad/1
  Compare To Constant/1 -> Switch/2
  Abs/1 -> Compare To Constant/1, Subtract/2
  psi_err_in/1 -> Abs/1, Switch/3, Sign/1

== system FMS/FMS Commander/Commander/Arm/Assist/Stabilize/Heading Command/Controller/Move Control/DeadZone ==
  u : Inport
  Dead Zone : DeadZone  LowerValue=-th  UpperValue=th  SaturateOnIntegerOverflow=on
  Gain : Gain  Gain=1/(1-th)
  y : Outport
  wires:
  Gain/1 -> y/1
  Dead Zone/1 -> Gain/1
  u/1 -> Dead Zone/1

== system FMS/FMS Commander/Commander/Arm/Auto/Mission/Mission_SubSystem/Velocity Commander/Lateral Acceleration/Included Angle ==
  vec1 : Inport
  vec2 : Inport  Port=2
  2D Cross Product : FMT_Model_Lib/Math/2D Cross Product
      settings: SourceProductName=FMT Toolbox
  Acos : Trigonometry  Operator=acos
  Constant4 : Constant  OutDataTypeStr=single
  Demux : Demux  Outputs=2
  Demux1 : Demux  Outputs=2
  Dot Product : DotProduct  InputSameDT=on  OutDataTypeStr=Inherit: Inherit via internal rule
  Multiply : Product
  Mux : Mux  Inputs=2
  Mux1 : Mux  Inputs=2
  Sign1 : Signum
  Switch2 : Switch  Criteria=u2 ~= 0
  Vector Normalize : FMT_Model_Lib/Math/Vector Normalize
      settings: SourceProductName=FMT Toolbox
  Vector Normalize1 : FMT_Model_Lib/Math/Vector Normalize
      settings: SourceProductName=FMT Toolbox
  angle_rad : Outport
  wires:
  Switch2/1 -> Multiply/2
  Acos/1 -> Multiply/1
  Mux/1 -> Vector Normalize1/1
  vec2/1 -> Demux/1
  Constant4/1 -> Switch2/3
  Demux/1 -> Mux/2
  vec1/1 -> Demux1/1
  Multiply/1 -> angle_rad/1
  2D Cross Product/1 -> Sign1/1
  Vector Normalize/1 -> 2D Cross Product/2, Dot Product/1
  Demux/2 -> Mux/1
  Vector Normalize1/1 -> 2D Cross Product/1, Dot Product/2
  Sign1/1 -> Switch2/2, Switch2/1
  Demux1/2 -> Mux1/1
  Mux1/1 -> Vector Normalize/1
  Demux1/1 -> Mux1/2
  Dot Product/1 -> Acos/1

== system FMS/FMS Commander/Commander/Arm/Auto/Offboard/Rotation_Command/Velocity Commander/Lateral Acceleration/Included Angle ==
  vec1 : Inport
  vec2 : Inport  Port=2
  2D Cross Product : FMT_Model_Lib/Math/2D Cross Product
      settings: SourceProductName=FMT Toolbox
  Acos : Trigonometry  Operator=acos
  Constant4 : Constant  OutDataTypeStr=single
  Demux : Demux  Outputs=2
  Demux1 : Demux  Outputs=2
  Dot Product : DotProduct  InputSameDT=on  OutDataTypeStr=Inherit: Inherit via internal rule
  Multiply : Product
  Mux : Mux  Inputs=2
  Mux1 : Mux  Inputs=2
  Sign1 : Signum
  Switch2 : Switch  Criteria=u2 ~= 0
  Vector Normalize : FMT_Model_Lib/Math/Vector Normalize
      settings: SourceProductName=FMT Toolbox
  Vector Normalize1 : FMT_Model_Lib/Math/Vector Normalize
      settings: SourceProductName=FMT Toolbox
  angle_rad : Outport
  wires:
  Switch2/1 -> Multiply/2
  Acos/1 -> Multiply/1
  Mux/1 -> Vector Normalize1/1
  vec2/1 -> Demux/1
  Constant4/1 -> Switch2/3
  Demux/1 -> Mux/2
  vec1/1 -> Demux1/1
  Multiply/1 -> angle_rad/1
  2D Cross Product/1 -> Sign1/1
  Vector Normalize/1 -> 2D Cross Product/2, Dot Product/1
  Demux/2 -> Mux/1
  Vector Normalize1/1 -> 2D Cross Product/1, Dot Product/2
  Sign1/1 -> Switch2/2, Switch2/1
  Demux1/2 -> Mux1/1
  Mux1/1 -> Vector Normalize/1
  Demux1/1 -> Mux1/2
  Dot Product/1 -> Acos/1

== system FMS/FMS Commander/Commander/Arm/Auto/Offboard/Rotation_Command/Way Points/Position_Control/Body_FRD ==
  psi : Inport
  pos_B_cmd : Inport  Port=2
  pos_mask : Inport  Port=3
  Data Store Read : DataStoreRead  DataStoreName=home
  Multiply : Product
  Multiply1 : Product  Multiplication=Matrix(*)
  Psi To DCM : FMT_Model_Lib/Transformation/Psi To DCM
      settings: SourceProductName=FMT Toolbox
  Selector1 : Selector  InputPortWidth=4  IndexOptions=Index vector (dialog)  Indices=[1:3]  OutputSizes=1
  Sum : Sum  Inputs=++|
  Transpose : Math  Operator=transpose  SaturateOnIntegerOverflow=on
  pos_O_cmd : Outport
  wires:
  Psi To DCM/1 -> Transpose/1
  psi/1 -> Psi To DCM/1
  Multiply/1 -> Multiply1/2
  pos_mask/1 -> Multiply/2
  Transpose/1 -> Multiply1/1  "M_OC"
  Data Store Read/1 -> Selector1/1
  pos_B_cmd/1 -> Multiply/1
  Multiply1/1 -> Sum/2
  Sum/1 -> pos_O_cmd/1
  Selector1/1 -> Sum/1

== system FMS/FMS Commander/Commander/Arm/Auto/Offboard/Rotation_Command/Way Points/Position_Control/Command_Mask ==
  FMS_In : Inport
  Bus Selector3 : BusSelector  OutputSignals=Auto_Cmd.cmd_mask
  Compare To Zero : simulink/Logic and Bit Operations/Compare To Zero  relop=>  OutDataTypeStr=boolean
  Compare To Zero1 : simulink/Logic and Bit Operations/Compare To Zero  relop=>  OutDataTypeStr=boolean
  Logical Operator : Logic  Operator=OR  AllPortsSameDT=off  OutDataTypeStr=boolean
  Mux : Mux  Inputs=3
  Mux3 : Mux  Inputs=3
  alt_cmd valid : simulink/Logic and Bit Operations/Bitwise Operator  logicop=AND  UseBitMask=on  BitMask=bin2dec('1000000000000')  BitMaskRealWorld=Stored Integer
  lat_cmd valid : simulink/Logic and Bit Operations/Bitwise Operator  logicop=AND  UseBitMask=on  BitMask=bin2dec('10000000000')  BitMaskRealWorld=Stored Integer
  lon_cmd valid : simulink/Logic and Bit Operations/Bitwise Operator  logicop=AND  UseBitMask=on  BitMask=bin2dec('100000000000')  BitMaskRealWorld=Stored Integer
  x_cmd valid : simulink/Logic and Bit Operations/Bitwise Operator  logicop=AND  UseBitMask=on  BitMask=bin2dec('10000000')  BitMaskRealWorld=Stored Integer
  y_cmd valid : simulink/Logic and Bit Operations/Bitwise Operator  logicop=AND  UseBitMask=on  BitMask=bin2dec('100000000')  BitMaskRealWorld=Stored Integer
  z_cmd valid : simulink/Logic and Bit Operations/Bitwise Operator  logicop=AND  UseBitMask=on  BitMask=bin2dec('1000000000')  BitMaskRealWorld=Stored Integer
  pos_mask : Outport
  wires:
  FMS_In/1 -> Bus Selector3/1
  x_cmd valid/1 -> Mux/1
  z_cmd valid/1 -> Mux/3
  y_cmd valid/1 -> Mux/2
  Mux/1 -> Compare To Zero/1
  lon_cmd valid/1 -> Mux3/2
  alt_cmd valid/1 -> Mux3/3
  Mux3/1 -> Compare To Zero1/1
  lat_cmd valid/1 -> Mux3/1
  Bus Selector3/1 -> y_cmd valid/1, x_cmd valid/1, z_cmd valid/1, lat_cmd valid/1, lon_cmd valid/1, alt_cmd valid/1  "<cmd_mask>"
  Compare To Zero1/1 -> Logical Operator/2
  Compare To Zero/1 -> Logical Operator/1
  Logical Operator/1 -> pos_mask/1

== system FMS/FMS Commander/Commander/Arm/Auto/Offboard/Rotation_Command/Way Points/Position_Control/Global_NED ==
  pos_O_cmd : Inport
  pos_mask : Inport  Port=2
  Multiply : Product
  Psi To DCM : FMT_Model_Lib/Transformation/Psi To DCM
      settings: SourceProductName=FMT Toolbox
  pos_cmd : Outport
  wires:
  pos_O_cmd/1 -> Multiply/1
  Multiply/1 -> pos_cmd/1
  pos_mask/1 -> Multiply/2

== system FMS/FMS Commander/Commander/Arm/Auto/Offboard/Rotation_Command/Way Points/Position_Control/Local_FRD ==
  pos_R_cmd : Inport
  pos_mask : Inport  Port=2
  Data Store Read : DataStoreRead  DataStoreName=home
  Multiply : Product
  Multiply3 : Product  Multiplication=Matrix(*)
  Psi To DCM2 : FMT_Model_Lib/Transformation/Psi To DCM
      settings: SourceProductName=FMT Toolbox
  Selector : Selector  InputPortWidth=4  IndexOptions=Index vector (dialog)  Indices=4  OutputSizes=1
  Selector1 : Selector  InputPortWidth=4  IndexOptions=Index vector (dialog)  Indices=[1:3]  OutputSizes=1
  Sum : Sum  Inputs=++|
  Transpose : Math  Operator=transpose  SaturateOnIntegerOverflow=on
  pos_O_cmd : Outport
  wires:
  Multiply/1 -> Multiply3/2
  pos_mask/1 -> Multiply/2
  Psi To DCM2/1 -> Transpose/1
  Transpose/1 -> Multiply3/1  "M_OC"
  Selector/1 -> Psi To DCM2/1
  Data Store Read/1 -> Selector/1, Selector1/1
  pos_R_cmd/1 -> Multiply/1
  Selector1/1 -> Sum/1
  Multiply3/1 -> Sum/2
  Sum/1 -> pos_O_cmd/1

== system FMS/FMS Commander/Commander/Arm/Auto/Offboard/Rotation_Command/Way Points/Position_Control/Local_NED ==
  pos_R_cmd : Inport
  pos_mask : Inport  Port=2
  Data Store Read : DataStoreRead  DataStoreName=home
  Multiply : Product
  Selector1 : Selector  InputPortWidth=4  IndexOptions=Index vector (dialog)  Indices=[1:3]  OutputSizes=1
  Sum : Sum  Inputs=++|
  pos_O_cmd : Outport
  wires:
  Sum/1 -> pos_O_cmd/1
  Selector1/1 -> Sum/1
  pos_R_cmd/1 -> Multiply/1
  Data Store Read/1 -> Selector1/1
  pos_mask/1 -> Multiply/2
  Multiply/1 -> Sum/2

== system FMS/FMS Commander/Commander/Arm/Auto/Offboard/Rotation_Command/Way Points/Position_Control/Position_Command ==
  FMS_In : Inport
  Command_Mask : Subsystem
  Global_Position_Command : Subsystem
  Local_Position_Command : Subsystem
  Switch : Switch  Criteria=u2 > Threshold
  pos_cmd_R : Outport
  wires:
  FMS_In/1 -> Local_Position_Command/1(FMS_In), Command_Mask/1(FMS_In), Global_Position_Command/1(FMS_In)
  Switch/1 -> pos_cmd_R/1
  Local_Position_Command/1(pos_cmd_R) -> Switch/3
  Global_Position_Command/1(pos_cmd_O) -> Switch/1
  Command_Mask/1(global_cmd_valid) -> Switch/2

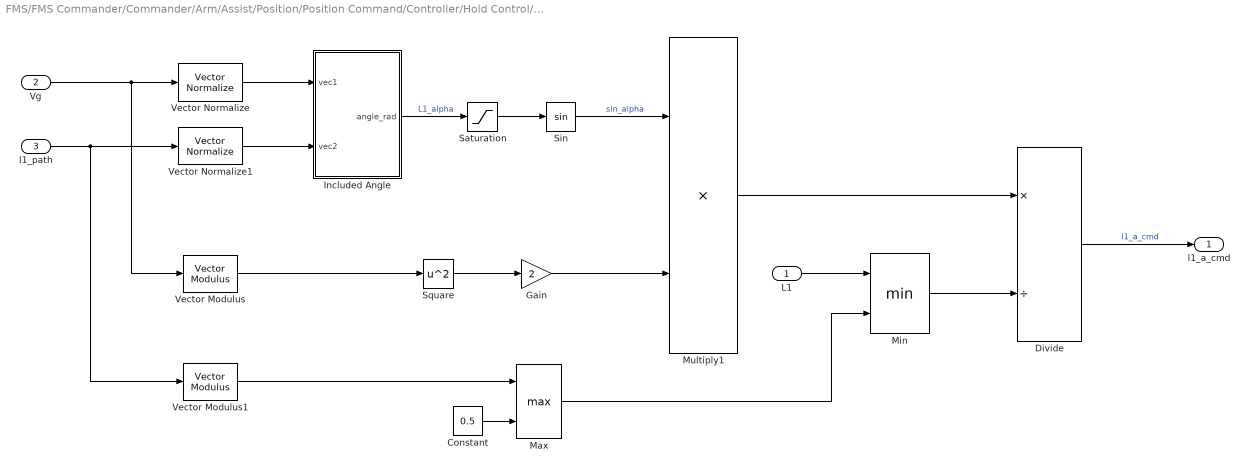
== system FMS/FMS Commander/Commander/Arm/Assist/Position/Position Command/Controller/Hold Control/Lateral_Acceleration/L1_Lateral_Acceleration ==
  L1 : Inport
  Vg : Inport  Port=2
  l1_path : Inport  Port=3
  Constant : Constant  Value=0.5  OutDataTypeStr=Inherit: Inherit via back propagation
  Divide : Product  Inputs=*/
  Gain : Gain  Gain=2
  Included Angle : Subsystem
  Max : MinMax  Function=max  Inputs=2
  Min : MinMax  Inputs=2
  Multiply1 : Product
  Saturation : Saturate  UpperLimit=pi/2  LowerLimit=-pi/2
  Sin : Trigonometry
  Square : Math  Operator=square  SaturateOnIntegerOverflow=on
  Vector Modulus : FMT_Model_Lib/Math/Vector Modulus
      settings: SourceProductName=FMT Toolbox
  Vector Modulus1 : FMT_Model_Lib/Math/Vector Modulus
      settings: SourceProductName=FMT Toolbox
  Vector Normalize : FMT_Model_Lib/Math/Vector Normalize
      settings: SourceProductName=FMT Toolbox
  Vector Normalize1 : FMT_Model_Lib/Math/Vector Normalize
      settings: SourceProductName=FMT Toolbox
  l1_a_cmd : Outport
  wires:
  Vector Normalize/1 -> Included Angle/1(vec1)
  Included Angle/1(angle_rad) -> Saturation/1  "L1_alpha"
  L1/1 -> Min/1
  Multiply1/1 -> Divide/1
  Divide/1 -> l1_a_cmd/1  "l1_a_cmd"
  Vector Normalize1/1 -> Included Angle/2(vec2)
  Sin/1 -> Multiply1/1  "sin_alpha"
  l1_path/1 -> Vector Modulus1/1, Vector Normalize1/1
  Saturation/1 -> Sin/1
  Vg/1 -> Vector Normalize/1, Vector Modulus/1
  Square/1 -> Gain/1
  Gain/1 -> Multiply1/2
  Min/1 -> Divide/2
  Max/1 -> Min/2
  Vector Modulus/1 -> Square/1
  Vector Modulus1/1 -> Max/1
  Constant/1 -> Max/2

== system FMS/FMS Commander/Commander/Arm/Assist/Position/Position Command/Controller/Hold Control/Path_Ray/sign ==
  u : Inport
  Constant : Constant  OutDataTypeStr=single
  Constant1 : Constant  Value=-1  OutDataTypeStr=single
  Switch : Switch
  s : Outport
  wires:
  u/1 -> Switch/2
  Switch/1 -> s/1
  Constant/1 -> Switch/1
  Constant1/1 -> Switch/3

== system FMS/FMS Commander/Commander/Arm/Auto/Offboard/Rotation_Command/Way Points/Position_Control/Position_Command/Command_Mask ==
  FMS_In : Inport
  Bus Selector3 : BusSelector  OutputSignals=Auto_Cmd.cmd_mask
  Compare To Zero : simulink/Logic and Bit Operations/Compare To Zero  relop=>  OutDataTypeStr=boolean
  Mux3 : Mux  Inputs=3
  alt_cmd valid : simulink/Logic and Bit Operations/Bitwise Operator  logicop=AND  UseBitMask=on  BitMask=bin2dec('1000000000000')  BitMaskRealWorld=Stored Integer
  lat_cmd valid : simulink/Logic and Bit Operations/Bitwise Operator  logicop=AND  UseBitMask=on  BitMask=bin2dec('10000000000')  BitMaskRealWorld=Stored Integer
  lon_cmd valid : simulink/Logic and Bit Operations/Bitwise Operator  logicop=AND  UseBitMask=on  BitMask=bin2dec('100000000000')  BitMaskRealWorld=Stored Integer
  global_cmd_valid : Outport
  wires:
  Bus Selector3/1 -> alt_cmd valid/1, lat_cmd valid/1, lon_cmd valid/1  "<cmd_mask>"
  lat_cmd valid/1 -> Mux3/1
  FMS_In/1 -> Bus Selector3/1
  Mux3/1 -> Compare To Zero/1
  lon_cmd valid/1 -> Mux3/2
  alt_cmd valid/1 -> Mux3/3
  Compare To Zero/1 -> global_cmd_valid/1

== system FMS/FMS Commander/Commander/Arm/Auto/Offboard/Rotation_Command/Way Points/Position_Control/Position_Command/Global_Position_Command ==
  FMS_In : Inport
  Bus Selector1 : BusSelector  OutputSignals=Auto_Cmd.lat_cmd,Auto_Cmd.lon_cmd,Auto_Cmd.alt_cmd
  Bus Selector2 : BusSelector  OutputSignals=INS_Out.lat_0,INS_Out.lon_0,INS_Out.alt_0
  Constant : Constant  Value=0
  Data Type Conversion : DataTypeConversion  OutDataTypeStr=double
  Data Type Conversion1 : DataTypeConversion  OutDataTypeStr=single
  Gain : Gain  Gain=1e-7  OutDataTypeStr=double
  Gain1 : Gain  Gain=1e-7  OutDataTypeStr=double
  Gain2 : Gain  Gain=-1
  LLA2FLAT : FMT_Model_Lib/Transformation/LLA2FLAT
      settings: SourceProductName=FMT Toolbox
  Mux : Mux  Inputs=3
  Mux1 : Mux  Inputs=2
  rad2deg : Gain  Gain=180/pi  OutDataTypeStr=double
  pos_cmd_O : Outport
  wires:
  Bus Selector1/3 -> Data Type Conversion/1  "<alt_cmd>"
  Gain/1 -> Mux/1
  Mux1/1 -> rad2deg/1
  Bus Selector1/1 -> Gain/1  "<lat_cmd>"
  FMS_In/1 -> Bus Selector2/1, Bus Selector1/1
  rad2deg/1 -> LLA2FLAT/2
  Gain1/1 -> Mux/2
  Bus Selector1/2 -> Gain1/1  "<lon_cmd>"
  Mux/1 -> LLA2FLAT/1
  Bus Selector2/1 -> Mux1/1  "<lat_0>"
  Data Type Conversion/1 -> Mux/3
  Bus Selector2/2 -> Mux1/2  "<lon_0>"
  LLA2FLAT/1 -> Data Type Conversion1/1
  Data Type Conversion1/1 -> pos_cmd_O/1
  Constant/1 -> LLA2FLAT/4
  Bus Selector2/3 -> Gain2/1  "<alt_0>"
  Gain2/1 -> LLA2FLAT/3

== system FMS/FMS Commander/Commander/Arm/Auto/Offboard/Rotation_Command/Way Points/Position_Control/Position_Command/Local_Position_Command ==
  FMS_In : Inport
  Bus Selector4 : BusSelector  OutputSignals=Auto_Cmd.x_cmd,Auto_Cmd.y_cmd,Auto_Cmd.z_cmd
  Mux2 : Mux  Inputs=3
  pos_cmd_R : Outport
  wires:
  Bus Selector4/1 -> Mux2/1  "<x_cmd>"
  Bus Selector4/2 -> Mux2/2  "<y_cmd>"
  FMS_In/1 -> Bus Selector4/1
  Bus Selector4/3 -> Mux2/3  "<z_cmd>"
  Mux2/1 -> pos_cmd_R/1  "pos_cmd"
